simulink library "Deadtime"  (R2026a)
settings: Solver=VariableStepAuto
undefined symbols (not defined in the file): deadtimeCfg, inverterCfg
settings Model: Creator=24322  LastModifiedBy=24322

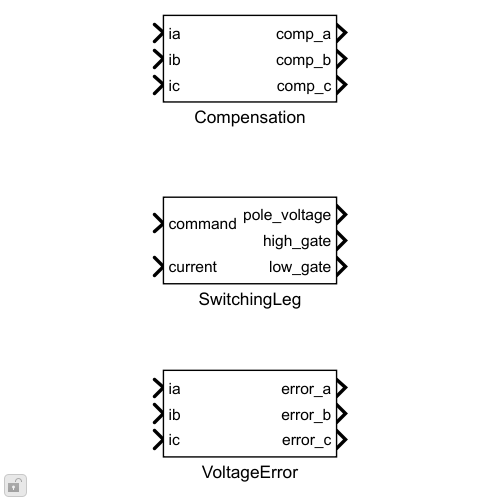
[thumbnail: Simulink's stored preview of the top-level diagram]
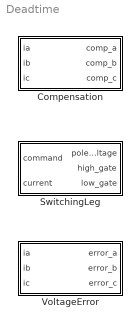
== system Deadtime ==
  Compensation : Subsystem
  SwitchingLeg : Subsystem
  VoltageError : Subsystem

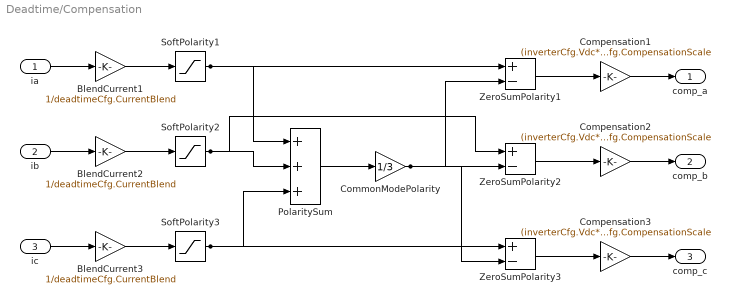
== system Deadtime/Compensation ==
  ia : Inport
  ib : Inport  Port=2
  ic : Inport  Port=3
  BlendCurrent1 : Gain  Gain=1/deadtimeCfg.CurrentBlend
  BlendCurrent2 : Gain  Gain=1/deadtimeCfg.CurrentBlend
  BlendCurrent3 : Gain  Gain=1/deadtimeCfg.CurrentBlend
  CommonModePolarity : Gain  Gain=1/3
  Compensation1 : Gain  Gain=(inverterCfg.Vdc*deadtimeCfg.DeadTime/inverterCfg.PwmTs+deadtimeCfg.DeviceDrop)*deadtimeCfg.CompensationEnable*deadtimeCfg.CompensationScale
  Compensation2 : Gain  Gain=(inverterCfg.Vdc*deadtimeCfg.DeadTime/inverterCfg.PwmTs+deadtimeCfg.DeviceDrop)*deadtimeCfg.CompensationEnable*deadtimeCfg.CompensationScale
  Compensation3 : Gain  Gain=(inverterCfg.Vdc*deadtimeCfg.DeadTime/inverterCfg.PwmTs+deadtimeCfg.DeviceDrop)*deadtimeCfg.CompensationEnable*deadtimeCfg.CompensationScale
  PolaritySum : Sum  Inputs=+++
  SoftPolarity1 : Saturate  UpperLimit=1  LowerLimit=-1
  SoftPolarity2 : Saturate  UpperLimit=1  LowerLimit=-1
  SoftPolarity3 : Saturate  UpperLimit=1  LowerLimit=-1
  ZeroSumPolarity1 : Sum  Inputs=+-
  ZeroSumPolarity2 : Sum  Inputs=+-
  ZeroSumPolarity3 : Sum  Inputs=+-
  comp_a : Outport
  comp_b : Outport  Port=2
  comp_c : Outport  Port=3
  wires:
  Compensation3/1 -> comp_c/1
  ZeroSumPolarity3/1 -> Compensation3/1
  SoftPolarity3/1 -> PolaritySum/3, ZeroSumPolarity3/1
  BlendCurrent3/1 -> SoftPolarity3/1
  ic/1 -> BlendCurrent3/1
  Compensation2/1 -> comp_b/1
  ZeroSumPolarity2/1 -> Compensation2/1
  SoftPolarity2/1 -> PolaritySum/2, ZeroSumPolarity2/1
  BlendCurrent2/1 -> SoftPolarity2/1
  ib/1 -> BlendCurrent2/1
  Compensation1/1 -> comp_a/1
  ZeroSumPolarity1/1 -> Compensation1/1
  CommonModePolarity/1 -> ZeroSumPolarity1/2, ZeroSumPolarity2/2, ZeroSumPolarity3/2
  SoftPolarity1/1 -> PolaritySum/1, ZeroSumPolarity1/1
  BlendCurrent1/1 -> SoftPolarity1/1
  ia/1 -> BlendCurrent1/1
  PolaritySum/1 -> CommonModePolarity/1

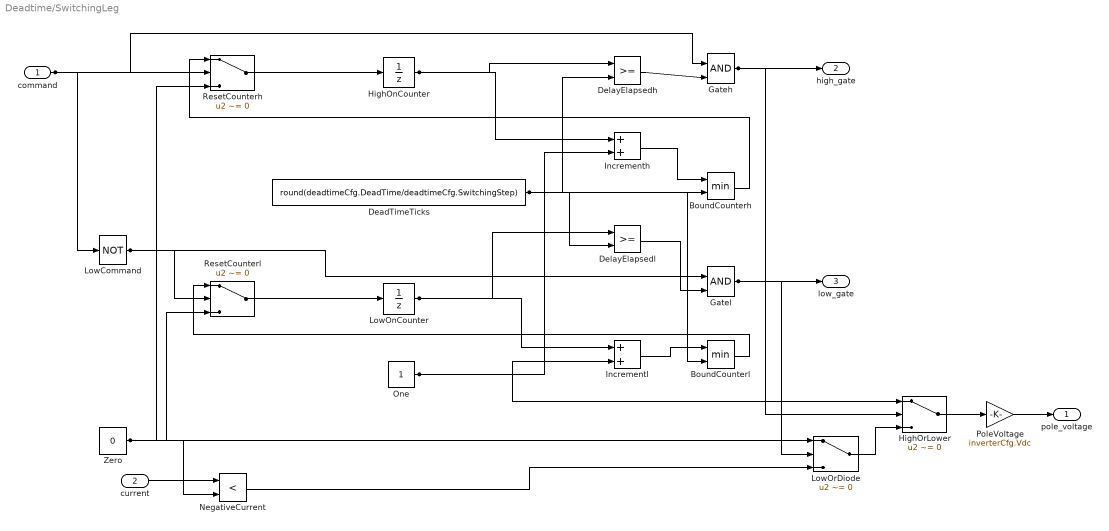
== system Deadtime/SwitchingLeg ==
  command : Inport
  current : Inport  Port=2
  BoundCounterh : MinMax  Inputs=2
  BoundCounterl : MinMax  Inputs=2
  DeadTimeTicks : Constant  Value=round(deadtimeCfg.DeadTime/deadtimeCfg.SwitchingStep)
  DelayElapsedh : RelationalOperator  OutDataTypeStr=boolean  RndMeth=Simplest  InputSameDT=off
  DelayElapsedl : RelationalOperator  OutDataTypeStr=boolean  RndMeth=Simplest  InputSameDT=off
  Gateh : Logic  IconShape=distinctive  AllPortsSameDT=off  OutDataTypeStr=boolean
  Gatel : Logic  IconShape=distinctive  AllPortsSameDT=off  OutDataTypeStr=boolean
  HighOnCounter : UnitDelay  SampleTime=deadtimeCfg.SwitchingStep
  HighOrLower : Switch  Criteria=u2 ~= 0  SaturateOnIntegerOverflow=off  InputSameDT=off
  Incrementh : Sum
  Incrementl : Sum
  LowCommand : Logic  Operator=NOT  IconShape=distinctive  AllPortsSameDT=off  OutDataTypeStr=boolean
  LowOnCounter : UnitDelay  SampleTime=deadtimeCfg.SwitchingStep
  LowOrDiode : Switch  Criteria=u2 ~= 0  SaturateOnIntegerOverflow=off  InputSameDT=off
  NegativeCurrent : RelationalOperator  Operator=<  OutDataTypeStr=boolean  RndMeth=Simplest  InputSameDT=off
  One : Constant
  PoleVoltage : Gain  Gain=inverterCfg.Vdc
  ResetCounterh : Switch  Criteria=u2 ~= 0  SaturateOnIntegerOverflow=off  InputSameDT=off
  ResetCounterl : Switch  Criteria=u2 ~= 0  SaturateOnIntegerOverflow=off  InputSameDT=off
  Zero : Constant  Value=0
  pole_voltage : Outport
  high_gate : Outport  Port=2
  low_gate : Outport  Port=3
  wires:
  PoleVoltage/1 -> pole_voltage/1
  HighOrLower/1 -> PoleVoltage/1
  LowOrDiode/1 -> HighOrLower/3
  Gateh/1 -> HighOrLower/2, high_gate/1
  NegativeCurrent/1 -> LowOrDiode/3
  Gatel/1 -> LowOrDiode/2, low_gate/1
  DelayElapsedl/1 -> Gatel/2
  ResetCounterl/1 -> LowOnCounter/1
  LowCommand/1 -> ResetCounterl/2, Gatel/1
  BoundCounterl/1 -> ResetCounterl/1
  Incrementl/1 -> BoundCounterl/1
  LowOnCounter/1 -> Incrementl/1, DelayElapsedl/1
  DelayElapsedh/1 -> Gateh/2
  ResetCounterh/1 -> HighOnCounter/1
  BoundCounterh/1 -> ResetCounterh/1
  DeadTimeTicks/1 -> BoundCounterh/2, BoundCounterl/2, DelayElapsedh/2, DelayElapsedl/2
  Incrementh/1 -> BoundCounterh/1
  One/1 -> HighOrLower/1, Incrementh/2, Incrementl/2
  HighOnCounter/1 -> Incrementh/1, DelayElapsedh/1
  Zero/1 -> LowOrDiode/1, NegativeCurrent/2, ResetCounterh/3, ResetCounterl/3
  current/1 -> NegativeCurrent/1
  command/1 -> LowCommand/1, ResetCounterh/2, Gateh/1

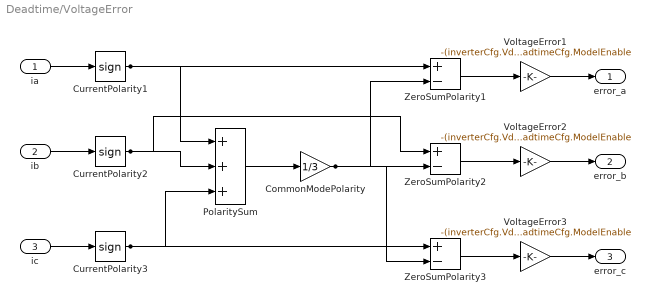
== system Deadtime/VoltageError ==
  ia : Inport
  ib : Inport  Port=2
  ic : Inport  Port=3
  CommonModePolarity : Gain  Gain=1/3
  CurrentPolarity1 : Signum
  CurrentPolarity2 : Signum
  CurrentPolarity3 : Signum
  PolaritySum : Sum  Inputs=+++
  VoltageError1 : Gain  Gain=-(inverterCfg.Vdc*deadtimeCfg.DeadTime/inverterCfg.PwmTs+deadtimeCfg.DeviceDrop)*deadtimeCfg.ModelEnable
  VoltageError2 : Gain  Gain=-(inverterCfg.Vdc*deadtimeCfg.DeadTime/inverterCfg.PwmTs+deadtimeCfg.DeviceDrop)*deadtimeCfg.ModelEnable
  VoltageError3 : Gain  Gain=-(inverterCfg.Vdc*deadtimeCfg.DeadTime/inverterCfg.PwmTs+deadtimeCfg.DeviceDrop)*deadtimeCfg.ModelEnable
  ZeroSumPolarity1 : Sum  Inputs=+-
  ZeroSumPolarity2 : Sum  Inputs=+-
  ZeroSumPolarity3 : Sum  Inputs=+-
  error_a : Outport
  error_b : Outport  Port=2
  error_c : Outport  Port=3
  wires:
  VoltageError3/1 -> error_c/1
  ZeroSumPolarity3/1 -> VoltageError3/1
  CurrentPolarity3/1 -> PolaritySum/3, ZeroSumPolarity3/1
  ic/1 -> CurrentPolarity3/1
  VoltageError2/1 -> error_b/1
  ZeroSumPolarity2/1 -> VoltageError2/1
  CurrentPolarity2/1 -> PolaritySum/2, ZeroSumPolarity2/1
  ib/1 -> CurrentPolarity2/1
  VoltageError1/1 -> error_a/1
  ZeroSumPolarity1/1 -> VoltageError1/1
  CommonModePolarity/1 -> ZeroSumPolarity1/2, ZeroSumPolarity2/2, ZeroSumPolarity3/2
  CurrentPolarity1/1 -> PolaritySum/1, ZeroSumPolarity1/1
  ia/1 -> CurrentPolarity1/1
  PolaritySum/1 -> CommonModePolarity/1
